simulink model "Main"  (Simulink 7.5)
settings: Solver=FixedStepDiscrete  StartTime=0.0  StopTime=Inf  FixedStep=0.001  RelTol=1e-3
undefined symbols (not defined in the file or in its folder): ecan1_buffered_transmit_matlab, ecan1_error_status_matlab, ecan1_init, ecan1_receive_matlab, u1, y1
libraries: simulink x20, dsPICdrivers x8
CloseFcn:
  | rtwprivate ssgencode ModelCloseRequest Main
settings Model: Creator=bwmairs  LastModifiedBy=bwmairs
settings OptimizationCC: InlineParams=on  InitFltsAndDblsToZero=on  OptimizeModelRefInitCode=on  LifeSpan=1
settings DebuggingCC: SaveWithParameterizedLinksMsg=none  StrictBusMsg=Warning
settings HardwareCC: ProdBitPerInt=16  ProdEndianess=LittleEndian  ProdWordSize=16  ProdHWDeviceType=16-bit Generic  TargetHWDeviceType=32-bit Generic
settings RTWCC: SystemTargetFile=dspic.tlc  TemplateMakefile=dspic_pic30_gcc.tmf  PostCodeGenCommand=dsPIC_Compile()  Description=Embedded Target for Microchip dsPIC (real-time)  ProcessScript=dspic_make_rtw_hook
settings RTWCC: CustomSource=|
  | ../../cBuffer.c
  | ../../ecanFunctions.c
  | ../../sbrk.c
settings CodeAppCC: IgnoreCustomStorageClasses=off
settings STFCustomTargetCC: TargetFcnLib=ansi_tfl_tmw.mat  IncludeMdlTerminateFcn=off  CombineOutputUpdateFcns=on  SuppressErrorStatus=on  ERTCustomFileBanners=on  SupportContinuousTime=off  SupportNonInlinedSFcns=off  CPPClassGenCompliant=on  SystemTargetFile=dspic.tlc
settings ERTTargetCC: TargetFcnLib=ansi_tfl_tmw.mat  MultiwordLength=2048  ParMdlRefBuildCompliant=off  CompOptLevelCompliant=off  IncludeMdlTerminateFcn=off  SuppressErrorStatus=on  ERTFirstTimeCompliant=off  ModelStepFunctionPrototypeControlCompliant=off  ExtModeMexFile=noextcomm  InlinedParameterPlacement=NonHierarchical  ERTSrcFileBannerTemplate=dsPIC_code_template.cgt  ERTHdrFileBannerTemplate=dsPIC_code_template.cgt  ERTDataSrcFileTemplate=dsPIC_code_template.cgt  ERTDataHdrFileTemplate=dsPIC_code_template.cgt  ERTCustomFileTemplate=dsPIC_main.tlc  ConvertIfToSwitch=off
settings CustomProperty: DataType=string  Value=C:\PROGRA~1\MATLAB\R2010a\bin\win32\gmake

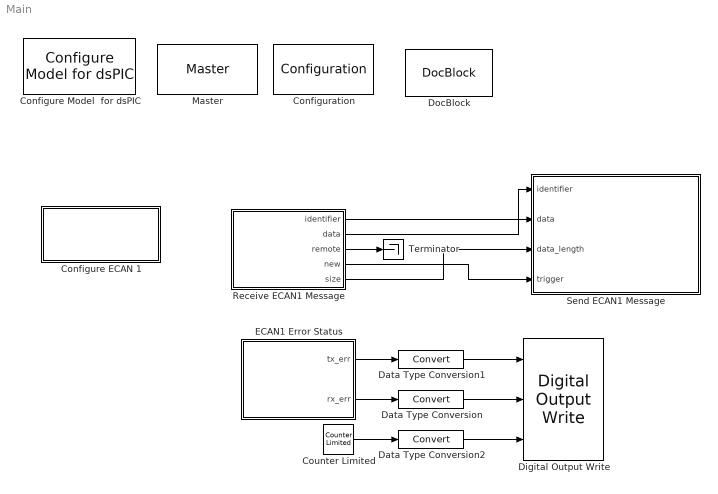
== system Main ==
  Configuration : dsPICdrivers/Configuration  SystemSampleTime=-1  double64=off
  Configure ECAN 1 : Subsystem  mask(Initialize ECAN 1){frame_setting=off, mode=Normal, dma_rx_chan=2, dma_tx_chan=0, baud=250000, ps1=8, pd=5, ps2=6, sjw=4, tq=20, triple_sample=on, dma_buf_size=4 buffers, rx_bufs=[1], tx_bufs=[0], buf_0_tx_pri=Highest, buf_0_rte=No, buf_1_tx_pri=Highest, buf_1_rte=No, buf_2_tx_pri=Lowest, buf_2_rte=No, buf_3_tx_pri=Lowest, buf_3_rte=No, buf_4_tx_pri=Lowest, buf_4_rte=No, buf_5_tx_pri=Lowest, buf_5_rte=No, buf_6_tx_pri=Lowest, buf_6_rte=No, buf_7_tx_pri=Lowest, buf_7_rte=No, mask_0=0, mask_0_mide=Match std or ext, mask_1=0, mask_1_mide=Match std or ext, mask_2=0, mask_2_mide=Match std or ext, filters=[0 1 2], filter_0=hex2dec('400'), filter_0_mask=0, filter_0_exide=Match only standard, filter_0_buf=1, filter_1=hex2dec('401'), filter_1_mask=0, filter_1_exide=Match only standard, filter_1_buf=1, filter_2=hex2dec('402'), filter_2_mask=0, filter_2_exide=Match only standard, filter_2_buf=1, filter_3=0, filter_3_mask=0, filter_3_exide=Match only standard, filter_3_buf=0, filter_4=0, filter_4_mask=0, filter_4_exide=Match only standard, filter_4_buf=0, filter_5=0, filter_5_mask=0, filter_5_exide=Match only standard, filter_5_buf=0, filter_6=0, filter_6_mask=0, filter_6_exide=Match only standard, filter_6_buf=0, filter_7=0, filter_7_mask=0, filter_7_exide=Match only standard, filter_7_buf=0, filter_8=0, filter_8_mask=0, filter_8_exide=Match only standard, filter_8_buf=0, filter_9=0, filter_9_mask=<empty>, filter_9_exide=Match only standard, filter_9_buf=0, filter_10=0, filter_10_mask=0, filter_10_exide=Match only standard, filter_10_buf=0, filter_11=0, filter_11_mask=0, filter_11_exide=Match only standard, filter_11_buf=0, filter_12=0, filter_12_mask=0, filter_12_exide=Match only standard, filter_12_buf=0, filter_13=0, filter_13_mask=0, filter_13_exide=Match only standard, filter_13_buf=0, filter_14=0, filter_14_mask=0, filter_14_exide=Match only standard, filter_14_buf=0, filter_15=0, filter_15_mask=0, filter_15_exide=Match only standard, filter_15_buf=0}
      mask prompts: frame_setting "Extended Frames (Standard if unchecked)"; dma_rx_chan "DMA Reception Channel"; dma_tx_chan "DMA Transmission Channel"; baud "Baud Rate (bps)"; ps1 "Phase Segment 1"; pd "Propagation Delay"; ps2 "Phase Segment 2"; sjw "Sync Jump Width"; tq "Time Quanta"; triple_sample "Triple-sample"; dma_buf_size "DMA Buffer Size"; rx_bufs "Reception Buffers"; tx_bufs "Transmission Buffers"; buf_0_tx_pri "Buffer 0 Transmission Priority"; buf_0_rte "Buffer 0 Remote Transmit Enable"; buf_1_tx_pri "Buffer 1 Transmission Priority"; buf_1_rte "Buffer 1 Remote Transmit Enable"; buf_2_tx_pri "Buffer 2 Transmission Priority"; buf_2_rte "Buffer 2 Remote Transmit Enable"; buf_3_tx_pri "Buffer 3 Transmission Priority"; buf_3_rte "Buffer 3 Remote Transmit Enable"; buf_4_tx_pri "Buffer 4 Transmission Priority"; buf_4_rte "Buffer 4 Remote Transmit Enable"; buf_5_tx_pri "Buffer 5 Transmission Priority"; buf_5_rte "Buffer 5 Remote Transmit Enable"; buf_6_tx_pri "Buffer 6 Transmission Priority"; buf_6_rte "Buffer 6 Remote Transmit Enable"; buf_7_tx_pri "Buffer 7 Transmission Priority"; buf_7_rte "Buffer 7 Remote Transmit Enable"; mask_0 "Mask 0"; mask_0_mide "Mask 0 Receive Mode"; mask_1 "Mask 1"; mask_1_mide "Mask 1 Receive Mode"; mask_2 "Mask 2"; mask_2_mide "Mask 2 Receive Mode"; filter_0 "Filter 0"; filter_0_mask "Filter 0 Mask"; filter_0_exide "Filter 0 Mode"; filter_0_buf "Filter 0 Buffer"; filter_1 "Filter 1"; filter_1_mask "Filter 1 Mask"; filter_1_exide "Filter 1 Mode"; filter_1_buf "Filter 1 Buffer"; filter_2 "Filter 2"; filter_2_mask "Filter 2 Mask"; filter_2_exide "Filter 2 Mode"; filter_2_buf "Filter 2 Buffer"; filter_3 "Filter 3"; filter_3_mask "Filter 3 Mask"; filter_3_exide "Filter 3 Mode"; filter_3_buf "Filter 3 Buffer"; filter_4 "Filter 4"; filter_4_mask "Filter 4 Mask"; filter_4_exide "Filter 4 Mode"; filter_4_buf "Filter 4 Buffer"; filter_5 "Filter 5"; filter_5_mask "Filter 5 Mask"; filter_5_exide "Filter 5 Mode"; filter_5_buf "Filter 5 Buffer"; filter_6 "Filter 6"; filter_6_mask "Filter 6 Mask"; filter_6_exide "Filter 6 Mode"; filter_6_buf "Filter 6 Buffer"; filter_7 "Filter 7"; filter_7_mask "Filter 7 Mask"; filter_7_exide "Filter 7 Mode"; filter_7_buf "Filter 7 Buffer"; filter_8 "Filter 8"; filter_8_mask "Filter 8 Mask"; filter_8_exide "Filter 8 Mode"; filter_8_buf "Filter 8 Buffer"; filter_9 "Filter 9"; filter_9_mask "Filter 9 Mask"; filter_9_exide "Filter 9 Mode"; filter_9_buf "Filter 9 Buffer"; filter_10 "Filter 10"; filter_10_mask "Filter 10 Mask"; filter_10_exide "Filter 10 Mode"; filter_10_buf "Filter 10 Buffer"; filter_11 "Filter 11"; filter_11_mask "Filter 11 Mask"; filter_11_exide "Filter 11 Mode"; filter_11_buf "Filter 11 Buffer"; filter_12 "Filter 12"; filter_12_mask "Filter 12 Mask"; filter_12_exide "Filter 12 Mode"; filter_12_buf "Filter 12 Buffer"; filter_13 "Filter 13"; filter_13_mask "Filter 13 Mask"; filter_13_exide "Filter 13 Mode"; filter_13_buf "Filter 13 Buffer"; filter_14 "Filter 14"; filter_14_mask "Filter 14 Mask"; filter_14_exide "Filter 14 Mode"; filter_14_buf "Filter 14 Buffer"; filter_15 "Filter 15"; filter_15_mask "Filter 15 Mask"; filter_15_exide "Filter 15 Mode"; filter_15_buf "Filter 15 Buffer"
      mask help: Initializes the ECAN 1 module on the dsPIC33f. Allows for configuration of almost all ECAN options to produce a usable system.
      mask init:
      | parameters = uint16(zeros(53,1));
      | 
      | %% Generate parameter 1
      | parameters(1) = frame_setting;
      | mode_id = 0;
      | switch mode
      |     case 'Disabled'
      |         mode_id = 1;
      |     case 'Loopback'
      |         mode_id = 2;
      |     case 'Listen only'
      |         mode_id = 3;
      |     case 'Listen all'
      |         mode_id = 7;
      | end
      | parameters(1) = bitor(parameters(1), bitshift(mode_id, 2));
      | parameters(1) = bitor(parameters(1), bitshift(dma_rx_chan, 5));
      | parameters(1) = bitor(parameters(1), bitshift(dma_tx_chan, 8));
      | 
      | %% Generate parameter 2
      | parameters(2) = baud / 100;
      | 
      | %% Generate parameter 3
      | h = find_system(bdroot(gcb),'FollowLinks','on','LookUnderMasks','all','Tag','dsPIC_MASTER');
      | fcy = 0;
      | if ~isempty(h)
      |     %OverrideFcy = strcmp(get_param(h{1},'OverrideFcy'),'on');
      |     %if (OverrideFcy == 1)
      |     %    fcy = str2num(get_param(h{1},'NewFcy'));     %% overridded fcy
      |     %else
      |         fcy = str2num(get_param(h{1},'fcy'));
      |     %end 
      | end
      | parameters(3) = fcy / 1000;
      | 
      | %% Generate parameter 4
      | parameters(4) = ps1 - 1;
      | parameters(4) = bitor(parameters(4), bitshift(pd - 1, 3));
      | parameters(4) = bitor(parameters(4), bitshift(ps2 - 1, 6));
      | parameters(4) = bitor(parameters(4), bitshift(sjw - 1, 9));
      | if triple_sample == 1
      |     parameters(4) = bitset(parameters(4),12);
      | end
      | 
      | %% Generate parameter 5
      | for k = 1:length(filters)
      |     parameters(5) = bitset(parameters(5),filters(k)+1);
      | end;
      | 
      | % Map filter mask values into proper values
      | filter_masks = [filter_0_mask; filter_1_mask; filter_2_mask; filter_3_mask; filter_4_mask; filter_5_mask; filter_6_mask; filter_7_mask; filter_8_mask; filter_9_mask; filter_10_mask; filter_11_mask; filter_12_mask; filter_13_mask; filter_14_mask; filter_15_mask;];
      | filter_masks = filter_masks - 2;
      | filter_masks(filter_masks == -1) = 3;
      | 
      | %% Generate parameters 6 and 7
      | for k = 1:length(filters);
      |     filter = filters(k) + 1;
      |     if filter < 9
      |         parameters(6) = bitor(parameters(6), bitshift(filter_masks(filter),2*(filter-1)));
      |     else
      |         parameters(7) = bitor(parameters(7), bitshift(filter_masks(filter),2*(filter-9)));
      |     end
      | end
      | 
      | % Generate parameters 8 and 9
      | parameters(8) = bitshift(bitand(mask_0,hex2dec('18000000')),-27); % EID17-16
      | parameters(8) = bitor(parameters(8), bitshift(bitand(mask_0,hex2dec('7FF')), 5)); % SID
      | parameters(8) = bitor(parameters(8), bitshift(mask_0_mide - 1, 3)); % MIDE
      | parameters(9) = bitshift(bitand(mask_0,hex2dec('7FFF800')),-11); % EID15-0
      | 
      | %% Generate parameters 10 and 11
      | parameters(10) = bitshift(bitand(mask_1,hex2dec('18000000')),-27); % EID17-16
      | parameters(10) = bitor(parameters(10), bitshift(bitand(mask_1,hex2dec('7FF')), 5)); % SID
      | parameters(10) = bitor(parameters(10), bitshift(mask_1_mide - 1, 3)); % MIDE
      | parameters(11) = bitshift(bitand(mask_1,hex2dec('7FFF800')),-11); % EID15-0
      | 
      | %% Generate parameters 12 and 13
      | parameters(12) = bitshift(bitand(mask_2,hex2dec('18000000')),-27); % EID17-16
      | parameters(12) = bitor(parameters(12), bitshift(bitand(mask_2,hex2dec('7FF')), 5)); % SID
      | parameters(12) = bitor(parameters(12), bitshift(mask_2_mide - 1, 3)); % MIDE
      | parameters(13) = bitshift(bitand(mask_2,hex2dec('7FFF800')),-11); % EID15-0
      | 
      | % Generate parameters 14-17
      | buf_priorities = [buf_0_tx_pri;buf_1_tx_pri;buf_2_tx_pri;buf_3_tx_pri;buf_4_tx_pri;buf_5_tx_pri;buf_6_tx_pri;buf_7_tx_pri] - 1;
      | buf_rtes = [buf_0_rte;buf_1_rte;buf_2_rte;buf_3_rte;buf_4_rte;buf_5_rte;buf_6_rte;buf_7_rte] - 1;
      | 
      | % Create a vector of chars to modify
      | regs = uint16(zeros(8,1));
      | 
      | % Go through all enabled transmission buffers setting appropriate bits
      | for b = 1:size(tx_bufs,1)
      |     
      |     index = tx_bufs(b) + 1;
      |     
      |     % Set transmission bit
      |     regs(index) = bitset(regs(index),8);
      | 
      |     % Set priority bits
      |     regs(index) = bitor(regs(index), buf_priorities(index));
      | 
      |     % Set remote transmit enable bits
      |     if buf_rtes(index) == 1
      |         regs(index) = bitset(regs(index),3);
      |     end
      | end
      | 
      | for b = 1:size(rx_bufs,1)
      |     
      |     index = rx_bufs(b) + 1;
      | 
      |     % Set priority bits
      |     regs(index) = bitor(regs(index), buf_priorities(index));
      | 
      |     % Set remote transmit enable bits
      |     if buf_rtes(index) == 1
      |         regs(index) = bitset(regs(index),3);
      |     end
      | end
      | 
      | % Map our matrix into registers
      | parameters(14) = bitor(bitshift(regs(2),8), regs(1));
      | parameters(15) = bitor(bitshift(regs(4),8), regs(3));
      | parameters(16) = bitor(bitshift(regs(6),8), regs(5));
      | parameters(17) = bitor(bitshift(regs(8),8), regs(7));
      | 
      | % Map the filter buffer values to corresponding bit values
      | filter_buffers = [filter_0_buf; filter_1_buf; filter_2_buf; filter_3_buf; filter_4_buf; filter_5_buf; filter_6_buf; filter_7_buf; filter_8_buf; filter_9_buf; filter_10_buf; filter_11_buf; filter_12_buf; filter_13_buf; filter_14_buf; filter_15_buf;];
      | filter_buffers = filter_buffers - 1;
      | 
      | %% Generate parameter 18
      | if bitget(parameters(5),1) == 1
      |     parameters(18) = filter_buffers(1);
      | end
      | if bitget(parameters(5),2) == 1
      |     parameters(18) = bitor(parameters(18), bitshift(filter_buffers(2), 4));
      | end
      | if bitget(parameters(5),3) == 1
      |     parameters(18) = bitor(parameters(18), bitshift(filter_buffers(3), 8));
      | end
      | if bitget(parameters(5),4) == 1
      |     parameters(18) = bitor(parameters(18), bitshift(filter_buffers(4), 12));
      | end
      | 
      | %% Generate parameter 19
      | if bitget(parameters(5),5) == 1
      |     parameters(19) = filter_buffers(5);
      | end
      | if bitget(parameters(5),6) == 1
      |     parameters(19) = bitor(parameters(19), bitshift(filter_buffers(6), 4));
      | end
      | if bitget(parameters(5),7) == 1
      |     parameters(19) = bitor(parameters(19), bitshift(filter_buffers(7), 8));
      | end
      | if bitget(parameters(5),8) == 1
      |     parameters(19) = bitor(parameters(19), bitshift(filter_buffers(8), 12));
      | end
      | 
      | %% Generate parameter 20
      | if bitget(parameters(5),9) == 1
      |     parameters(20) = filter_buffers(9);
      | end
      | if bitget(parameters(5),10) == 1
      |     parameters(20) = bitor(parameters(20), bitshift(filter_buffers(10), 4));
      | end
      | if bitget(parameters(5),11) == 1
      |     parameters(20) = bitor(parameters(20), bitshift(filter_buffers(11), 8));
      | end
      | if bitget(parameters(5),12) == 1
      |     parameters(20) = bitor(parameters(20), bitshift(filter_buffers(12), 12));
      | end
      | 
      | %% Generate parameter 21
      | if bitget(parameters(5),13) == 1
      |     parameters(21) = filter_buffers(13);
      | end
      | if bitget(parameters(5),14) == 1
      |     parameters(21) = bitor(parameters(21), bitshift(filter_buffers(14), 4));
      | end
      | if bitget(parameters(5),15) == 1
      |     parameters(21) = bitor(parameters(21), bitshift(filter_buffers(15), 8));
      | end
      | if bitget(parameters(5),16) == 1
      |     parameters(21) = bitor(parameters(21), bitshift(filter_buffers(16), 12));
      | end
      | 
      | % Generate parameters 22 and 23
      | parameters(22) = bitshift(bitand(filter_0,hex2dec('18000000')),-27); % EID17-16
      | parameters(22) = bitor(parameters(22), bitshift(bitand(filter_0,hex2dec('7FF')), 5)); % SID
      | parameters(22) = bitor(parameters(22), bitshift(filter_0_exide - 1, 3)); % EXIDE
      | parameters(23) = bitshift(bitand(uint32(filter_0),hex2dec('7FFF800')),-11); % EID15-0
      | 
      | %% Generate parameters 24 and 25
      | parameters(24) = bitshift(bitand(filter_1,hex2dec('18000000')),-27); % EID17-16
      | parameters(24) = bitor(parameters(24), bitshift(bitand(filter_1,hex2dec('7FF')), 5)); % SID
      | parameters(24) = bitor(parameters(24), bitshift(filter_1_exide - 1, 3)); % EXIDE
      | parameters(25) = bitshift(bitand(uint32(filter_1),hex2dec('7FFF800')),-11); % EID15-0
      | 
      | %% Generate parameters 26 and 27
      | parameters(26) = bitshift(bitand(filter_2,hex2dec('18000000')),-27); % EID17-16
      | parameters(26) = bitor(parameters(26), bitshift(bitand(filter_2,hex2dec('7FF')), 5)); % SID
      | parameters(26) = bitor(parameters(26), bitshift(filter_2_exide - 1, 3)); % EXIDE
      | parameters(27) = bitshift(bitand(uint32(filter_2),hex2dec('7FFF800')),-11); % EID15-0
      | 
      | %% Generate parameters 28 and 29
      | parameters(28) = bitshift(bitand(filter_3,hex2dec('18000000')),-27); % EID17-16
      | parameters(28) = bitor(parameters(28), bitshift(bitand(filter_3,hex2dec('7FF')), 5)); % SID
      | parameters(28) = bitor(parameters(28), bitshift(filter_3_exide - 1, 3)); % EXIDE
      | parameters(29) = bitshift(bitand(uint32(filter_3),hex2dec('7FFF800')),-11); % EID15-0
      | 
      | %% Generate parameters 30 and 31
      | parameters(30) = bitshift(bitand(filter_4,hex2dec('18000000')),-27); % EID17-16
      | parameters(30) = bitor(parameters(30), bitshift(bitand(filter_4,hex2dec('7FF')), 5)); % SID
      | parameters(30) = bitor(parameters(30), bitshift(filter_4_exide - 1, 3)); % EXIDE
      | parameters(31) = bitshift(bitand(uint32(filter_4),hex2dec('7FFF800')),-11); % EID15-0
      | 
      | %% Generate parameters 32 and 33
      | parameters(32) = bitshift(bitand(filter_5,hex2dec('18000000')),-27); % EID17-16
      | parameters(32) = bitor(parameters(32), bitshift(bitand(filter_5,hex2dec('7FF')), 5)); % SID
      | parameters(32) = bitor(parameters(32), bitshift(filter_5_exide - 1, 3)); % EXIDE
      | parameters(33) = bitshift(bitand(uint32(filter_5),hex2dec('7FFF800')),-11); % EID15-0
      | 
      | %% Generate parameters 34 and 35
      | parameters(34) = bitshift(bitand(filter_6,hex2dec('18000000')),-27); % EID17-16
      | parameters(34) = bitor(parameters(34), bitshift(bitand(filter_6,hex2dec('7FF')), 5)); % SID
      | parameters(34) = bitor(parameters(34), bitshift(filter_6_exide - 1, 3)); % EXIDE
      | parameters(35) = bitshift(bitand(uint32(filter_6),hex2dec('7FFF800')),-11); % EID15-0
      | 
      | %% Generate parameters 36 and 37
      | parameters(36) = bitshift(bitand(filter_7,hex2dec('18000000')),-27); % EID17-16
      | parameters(36) = bitor(parameters(36), bitshift(bitand(filter_7,hex2dec('7FF')), 5)); % SID
      | parameters(36) = bitor(parameters(36), bitshift(filter_7_exide - 1, 3)); % EXIDE
      | parameters(37) = bitshift(bitand(uint32(filter_7),hex2dec('7FFF800')),-11); % EID15-0
      | 
      | %% Generate parameters 38 and 39
      | parameters(38) = bitshift(bitand(filter_8,hex2dec('18000000')),-27); % EID17-16
      | parameters(38) = bitor(parameters(38), bitshift(bitand(filter_8,hex2dec('7FF')), 5)); % SID
      | parameters(38) = bitor(parameters(38), bitshift(filter_8_exide - 1, 3)); % EXIDE
      | parameters(39) = bitshift(bitand(uint32(filter_8),hex2dec('7FFF800')),-11); % EID15-0
      | 
      | %% Generate parameters 40 and 41
      | parameters(40) = bitshift(bitand(filter_9,hex2dec('18000000')),-27); % EID17-16
      | parameters(40) = bitor(parameters(40), bitshift(bitand(filter_9,hex2dec('7FF')), 5)); % SID
      | parameters(40) = bitor(parameters(40), bitshift(filter_9_exide - 1, 3)); % EXIDE
      | parameters(41) = bitshift(bitand(uint32(filter_9),hex2dec('7FFF800')),-11); % EID15-0
      | 
      | %% Generate parameters 42 and 43
      | parameters(42) = bitshift(bitand(filter_10,hex2dec('18000000')),-27); % EID17-16
      | parameters(42) = bitor(parameters(42), bitshift(bitand(filter_10,hex2dec('7FF')), 5)); % SID
      | parameters(42) = bitor(parameters(42), bitshift(filter_10_exide - 1, 3)); % EXIDE
      | parameters(43) = bitshift(bitand(uint32(filter_10),hex2dec('7FFF800')),-11); % EID15-0
      | 
      | %% Generate parameters 44 and 45
      | parameters(44) = bitshift(bitand(filter_11,hex2dec('18000000')),-27); % EID17-16
      | parameters(44) = bitor(parameters(44), bitshift(bitand(filter_11,hex2dec('7FF')), 5)); % SID
      | parameters(44) = bitor(parameters(44), bitshift(filter_11_exide - 1, 3)); % EXIDE
      | parameters(45) = bitshift(bitand(uint32(filter_11),hex2dec('7FFF800')),-11); % EID15-0
      | 
      | %% Generate parameters 46 and 47
      | parameters(46) = bitshift(bitand(filter_12,hex2dec('18000000')),-27); % EID17-16
      | parameters(46) = bitor(parameters(46), bitshift(bitand(filter_12,hex2dec('7FF')), 5)); % SID
      | parameters(46) = bitor(parameters(46), bitshift(filter_12_exide - 1, 3)); % EXIDE
      | parameters(47) = bitshift(bitand(uint32(filter_12),hex2dec('7FFF800')),-11); % EID15-0
      | 
      | %% Generate parameters 48 and 49
      | parameters(48) = bitshift(bitand(filter_13,hex2dec('18000000')),-27); % EID17-16
      | parameters(48) = bitor(parameters(48), bitshift(bitand(filter_13,hex2dec('7FF')), 5)); % SID
      | parameters(48) = bitor(parameters(48), bitshift(filter_13_exide - 1, 3)); % EXIDE
      | parameters(49) = bitshift(bitand(uint32(filter_13),hex2dec('7FFF800')),-11); % EID15-0
      | 
      | %% Generate parameters 50 and 51
      | parameters(50) = bitshift(bitand(filter_14,hex2dec('18000000')),-27); % EID17-16
      | parameters(50) = bitor(parameters(50), bitshift(bitand(filter_14,hex2dec('7FF')), 5)); % SID
      | parameters(50) = bitor(parameters(50), bitshift(filter_14_exide - 1, 3)); % EXIDE
      | parameters(51) = bitshift(bitand(uint32(filter_14),hex2dec('7FFF800')),-11); % EID15-0
      | 
      | %% Generate parameters 52 and 53
      | parameters(52) = bitshift(bitand(filter_15,hex2dec('18000000')),-27); % EID17-16
      | parameters(52) = bitor(parameters(52), bitshift(bitand(filter_15,hex2dec('7FF')), 5)); % SID
      | parameters(52) = bitor(parameters(52), bitshift(filter_15_exide - 1, 3)); % EXIDE
      | parameters(53) = bitshift(bitand(uint32(filter_15),hex2dec('7FFF800')),-11); % EID15-0
      mask StyleString: checkbox,popup(Disabled|Listen all|Listen only|Loopback|Normal),edit,edit,edit,edit,edit,edit,popup(1|2|3|4),edit,checkbox,popup(4 buffers|6 buffers|8 buffers|12 buffers|16 buffers|24 buffers|32 buffers),edit,edit,popup(Lowest|Low|High|Highest),popup(No|Yes),popup(Lowest|Low|High|Highest),popup(No|Yes),popup(Lowest|Low|High|Highest),popup(No|Yes),popup(Lowest|Low|High|Highest),popup(No|Yes),popup(Lowest|Low|High|Highest),popup(No|Yes),popup(Lowest|Low|High|Highest),popup(No|Yes),popup(Lowest|Low|High|Highest),popup(No|Yes),popup(Lowest|Low|High|Highest),popup(No|Yes),edit,popup(Match std or ext|Obey filter mode),edit,popup(Match std or ext|Obey filter mode),edit,popup(Match std or ext|Obey filter mode),edit,edit,popup(--|0|1|2),popup(Match only standard|Match only extended),popup(0|1|2|3|4|5|6|7|8|9|10|11|12|13|14|FIFO),edit,popup(--|0|1|2),popup(Match only standard|Match only extended),popup(0|1|2|3|4|5|6|7|8|9|10|11|12|13|14|FIFO),edit,popup(--|0|1|2),popup(Match only standard|Match only extended),popup(0|1|2|3|4|5|6|7|8|9|10|11|12|13|14|FIFO),edit,popup(--|0|1|2),popup(Match only standard|Match only extended),popup(0|1|2|3|4|5|6|7|8|9|10|11|12|13|14|FIFO),edit,popup(--|0|1|2),popup(Match only standard|Match only extended),popup(0|1|2|3|4|5|6|7|8|9|10|11|12|13|14|FIFO),edit,popup(--|0|1|2),popup(Match only standard|Match only extended),popup(0|1|2|3|4|5|6|7|8|9|10|11|12|13|14|FIFO),edit,popup(--|0|1|2),popup(Match only standard|Match only extended),popup(0|1|2|3|4|5|6|7|8|9|10|11|12|13|14|FIFO),edit,popup(--|0|1|2),popup(Match only standard|Match only extended),popup(0|1|2|3|4|5|6|7|8|9|10|11|12|13|14|FIFO),edit,popup(--|0|1|2),popup(Match only standard|Match only extended),popup(0|1|2|3|4|5|6|7|8|9|10|11|12|13|14|FIFO),edit,popup(<empty>),popup(Match only standard|Match only extended),popup(0|1|2|3|4|5|6|7|8|9|10|11|12|13|14|FIFO),edit,popup(--|0|1|2),popup(Match only standard|Match only extended),popup(0|1|2|3|4|5|6|7|8|9|10|11|12|13|14|FIFO),edit,popup(--|0|1|2),popup(Match only standard|Match only extended),popup(0|1|2|3|4|5|6|7|8|9|10|11|12|13|14|FIFO),edit,popup(--|0|1|2),popup(Match only standard|Match only extended),popup(0|1|2|3|4|5|6|7|8|9|10|11|12|13|14|FIFO),edit,popup(--|0|1|2),popup(Match only standard|Match only extended),popup(0|1|2|3|4|5|6|7|8|9|10|11|12|13|14|FIFO),edit,popup(--|0|1|2),popup(Match only standard|Match only extended),popup(0|1|2|3|4|5|6|7|8|9|10|11|12|13|14|FIFO),edit,popup(--|0|1|2),popup(Match only standard|Match only extended),popup(0|1|2|3|4|5|6|7|8|9|10|11|12|13|14|FIFO)
      mask CallbackString:
      | |||||tq = 1 + str2num(get_param(gcb, 'ps1')) + str2num(get_param(gcb, 'pd')) + str2num(get_param(gcb, 'ps2'));
      | set_param(gcb, 'tq', int2str(tq));|tq = 1 + str2num(get_param(gcb, 'ps1')) + str2num(get_param(gcb, 'pd')) + str2num(get_param(gcb, 'ps2'));
      | set_param(gcb, 'tq', int2str(tq));|tq = 1 + str2num(get_param(gcb, 'ps1')) + str2num(get_param(gcb, 'pd')) + str2num(get_param(gcb, 'ps2'));
      | set_param(gcb, 'tq', int2str(tq));||||||filters = eval(get_param(gcb,'tx_bufs'));
      | mVisibilities = get_param(gcb,'MaskVisibilities');
      | mNames = get_param(gcb,'MaskNames');
      | for i = 1:size(mNames);
      | 	n = mNames{i};
      |     if size(n,2) > 4 && strcmp(n(1:4), 'buf_') == 1
      |         filterNumber = sscanf(n, 'buf_%d');
      |         if isempty(find(filters == filterNumber, 1)) == 0
      |              mVisibilities{i} = 'on';
      |         else
      |              mVisibilities{i} = 'off';
      |         end
      |     end
      | end
      | set_param(gcb, 'MaskVisibilities', mVisibilities);|||||||||||||||||||||||filters = eval(get_param(gcb,'filters'));
      | mVisibilities = get_param(gcb,'MaskVisibilities');
      | mNames = get_param(gcb,'MaskNames');
      | for i = 1:size(mNames);
      | 	n = mNames{i};
      |     if size(n,2) > 7 && strcmp(n(1:7), 'filter_') == 1
      |         filterNumber = sscanf(n, 'filter_%d');
      |         if isempty(find(filters == filterNumber, 1)) == 0
      |              mVisibilities{i} = 'on';
      |         else
      |              mVisibilities{i} = 'off';
      |         end
      |     end
      | end
      | set_param(gcb, 'MaskVisibilities', mVisibilities);||||||||||||||||||||||||||||||||||||||||||||||||||||||||||||||||
      mask Display: text(0.5,0.5,'Configure ECAN1','horizontalAlignment','center','verticalAlignment','middle');
  Configure Model  for dsPIC : dsPICdrivers/Simulink Configuration/Configure Model  for dsPIC
  Counter Limited : simulink/Sources/Counter Limited  SystemSampleTime=-1  uplimit=1  tsamp=.1
  Data Type Conversion : DataTypeConversion  OutDataType=sfix(16)  OutScaling=2^0
  Data Type Conversion1 : DataTypeConversion  OutDataType=sfix(16)  OutScaling=2^0
  Data Type Conversion2 : DataTypeConversion  OutDataType=sfix(16)  OutScaling=2^0
  Digital Output Write : dsPICdrivers/Digital I//O/Digital Output Write  Tag=dsPIC_Digital_Output  Priority=5  PORT=A  Pin=[0 1 7]  Simultaneous=off  OrderingInOutPopup=None
  DocBlock : simulink/Model-Wide Utilities/DocBlock  SystemSampleTime=-1  DocumentType=Text
      content=|
      | This model recreates the Crosswire application note from Microchip.
      | The Debugging directory includes an MPLAB project that can compile and load
      | the MATLAB-generated code in order to facilitate debugging.
  ECAN1 Error Status : Subsystem  mask(ECAN 1 Reception Block){ecan1_error_sample_time=.1}
      mask prompts: ecan1_error_sample_time "Sampling time"
      mask help:
      | This block will receive CAN messages over the ECAN1 peripheral on the dsPIC33f.
      | Outputs:
      | identifier - uint32 containing SID and EID
      | data - Variable-sized array (between 0 and 8) of uint8s
      | remote - boolean value specifying if this is a remote transmit request
      mask Display: disp('ECAN1 ERR');
  Master : dsPICdrivers/Master  Tag=dsPIC_MASTER  Priority=1  TimeStepType=Timer1  picType=choose_dsPIC_Target  fcy=5e6  Quartz_33f=5e6  PLLActive_33f=off  fcyDesired_33f=0  tmr1="[1  4999  0]"  tmr1Info="Time Step : 0.001  ;   Error : 0%  PR1=4999"  tmr2345="[0  0  0  0  0  0  0  0]"  tmr2345cfg=[-1 -1 -1 -1 -1 -1 -1 -1]  IOautoConf=on  typePort="[ 10  10   0   0   0   0   0  10   0   0   0   0   0   0   0   0   0   0   0   0   0   0   0   0   0   0   0   0   0   0   0   0   0   0   0   0   0   0   0   0   0   0   0   0   0   0   0   0   0   0   0   0   0   0   0   0   0   0   0   0   0   0   0   0   0   0   0   0   0   0   0   0   0   0   0   0   0   0   0   0   0   0   0   0   0   0   0   0   0   0   0   0   0   0   0   0   0   0   0   0   0   0   0   0   0   0   0   0   0   0   0   0 ]"  TRIS="[ 65404  65535  65535  65535  65535  65535  65535 ]"  ADPCFG=131  MasterBusyPort=None  MasterOverloadPort=None  FOSC=CSW_FSCM_OFF  ClockSwitchMonitor=Both disabled  TempProtection_33f=TEMP_ON  FPBOR=PBOR_OFF  PWRT=PWRT_OFF  MCLR=MCLR_DIS  ICD=ICS_NONE  JTAGEN=JTAGEN_OFF  PowerSave=off  OverrideFcy=off  NewFcy=1e6  PR2345="[65535  65535  65535  65535  65535  65535  65535  65535]"
  Receive ECAN1 Message : Subsystem  mask(ECAN 1 Reception Block){ecan1_receive_sample_time=.01}
      mask prompts: ecan1_receive_sample_time "Sampling time"
      mask help:
      | This block will receive CAN messages over the ECAN1 peripheral on the dsPIC33f.
      | Outputs:
      | identifier - uint32 containing SID and EID
      | data - Variable-sized array (between 0 and 8) of uint8s
      | remote - boolean value specifying if this is a remote transmit request
      mask Display: disp('ECAN1 RX');
  Send ECAN1 Message : Subsystem  Tag=dsPIC_MASTER  mask(Send ECAN Message){buffer=0, identifier=hex2dec('401'), identifier_from_input=on, ide=off, remote=off, data=[hex2dec('11') hex2dec('12') hex2dec('13') hex2dec('14')], data_length=4, data_from_input=on, c_func_sample_time=.01, trigger_on_input=on}
      mask prompts: identifier_from_input "Identifier from input"; data_length "Data length"; data_from_input "Data from input"; c_func_sample_time "Sample time"; trigger_on_input "Trigger on input"
      mask help: This block allows for the transmission of a message over the ECAN module.
      mask CallbackString:
      | ||mEnables = get_param(gcb,'MaskEnables');
      | enabled = get_param(gcb, 'identifier_from_input');
      | if strcmp(enabled,'on');
      |     replace_block([gcb '/identifier'],'Constant','Inport','noprompt');
      |     mEnables{2} = 'off';
      |     set_param([gcb '/identifier'],'Port','1');
      | else
      |     replace_block([gcb '/identifier'],'Inport','Constant','noprompt');
      |     mEnables{2} = 'on';
      |     set_param([gcb '/identifier'],'Value','identifier');
      | end
      | set_param(gcb, 'MaskEnables', mEnables);
      | |||data = eval(get_param(gcb, 'data'));
      | y = size(data,1);
      | x = size(data,2);
      | if y > 1 && x > 1
      |     error('Data must be a 1-dimensional vector')
      | else
      |     if or(x > 8, y > 8)
      |         error('Data cannot be larger than 8-bytes');
      |     end
      | end
      | 
      | set_param(gcb, 'data_length', num2str(length(data)));|data_length = eval(get_param(gcb, 'data_length'));
      | if or(data_length < 0, data_length > 9)
      |     error('Data cannot be more than 8 bytes or less than 0.')
      | end|mEnables = get_param(gcb,'MaskEnables');
      | enabled = get_param(gcb, 'data_from_input');
      | if strcmp(enabled,'on');
      |     replace_block([gcb '/data'],'Constant','Inport','noprompt');
      |     replace_block([gcb '/data_length'],'Constant','Inport','noprompt');
      |     mEnables{6} = 'off';
      |     mEnables{7} = 'off';
      |     port = 1;
      |     if ~isempty(find_system(gcb,'LookUnderMasks','all','Name','identifier'))
      |         port = 2;
      |     end
      |     set_param([gcb '/data'],'Port',num2str(port));
      |     set_param([gcb '/data_length'],'Port',num2str(port+1));
      | else
      |     replace_block([gcb '/data'],'Inport','Constant','noprompt');
      |     replace_block([gcb '/data_length'],'Inport','Constant','noprompt');
      |     mEnables{6} = 'on';
      |     mEnables{7} = 'on';
      |     set_param([gcb '/data'],'Value','data');
      |     set_param([gcb '/data'],'OutDataTypeMode','uint8');
      |     set_param([gcb '/data_length'],'Value','data_length');
      |     set_param([gcb '/data_length'],'OutDataTypeMode','uint8');
      | end
      | set_param(gcb, 'MaskEnables', mEnables);
      | ||mEnables = get_param(gcb,'MaskEnables');
      | enabled = get_param(gcb, 'trigger_on_input');
      | c_func_blk = find_system(gcb,'LookUnderMasks','all','FunctionName','dsPIC_C_function_Call');
      | if strcmp(enabled,'on');
      |     mEnables{9} = 'off';
      |     %set_param(c_func_blk,'SampleTime','-1');
      |     replace_block([gcb '/trigger'],'Constant','Inport','noprompt');
      | else
      |     mEnables{9} = 'on';
      |     %set_param(c_func_blk,'SampleTime','c_func_sample_time');
      |     replace_block([gcb '/trigger'],'Inport','Constant','noprompt');
      |     %set_param([gcb '/trigger'],'Value','1');
      | end
      | set_param(gcb, 'MaskEnables', mEnables);
      mask Display: disp('ECAN1 TX');
  Terminator : Terminator
  wires:
  Receive ECAN1 Message/3(remote) -> Terminator/1
  ECAN1 Error Status/2(rx_err) -> Data Type Conversion/1
  ECAN1 Error Status/1(tx_err) -> Data Type Conversion1/1
  Counter Limited/1 -> Data Type Conversion2/1
  Data Type Conversion1/1 -> Digital Output Write/1
  Data Type Conversion/1 -> Digital Output Write/2
  Data Type Conversion2/1 -> Digital Output Write/3
  Receive ECAN1 Message/2(data) -> Send ECAN1 Message/2(data)
  Receive ECAN1 Message/4(new) -> Send ECAN1 Message/4(trigger)
  Receive ECAN1 Message/5(size) -> Send ECAN1 Message/3(data_length)
  Receive ECAN1 Message/1(identifier) -> Send ECAN1 Message/1(identifier)

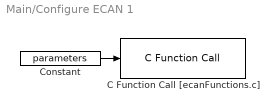
== system Main/Configure ECAN 1 ==
  C Function Call [ecanFunctions.c] : dsPICdrivers/OTHERS/C Function Call  Tag=dsPIC_dsPIC_CFunctionCall  fctName='ecan1_init'  INPUT_SIZE=53  INPUT1=uint16  INPUT2=--  INPUT3=--  OUTPUT_SIZE=1  OUTPUT1=--  SampleTime=Inf  InputType=[ 4 ]  OutputType=[ ]  FctDeclaration=extern void ecan1_init(uint16_T* u1);  FctCall=ecan1_init(*%u1);  OrderingInOutPopup=None
  Constant : Constant  Value=parameters  OutDataTypeMode=uint16  OutDataType=sfix(16)  OutScaling=2^0  OutDataTypeStr=uint16
  wires:
  Constant/1 -> C Function Call [ecanFunctions.c]/1

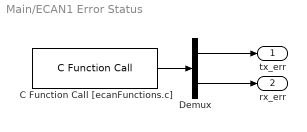
== system Main/ECAN1 Error Status ==
  C Function Call [ecanFunctions.c] : dsPICdrivers/OTHERS/C Function Call  Tag=dsPIC_dsPIC_CFunctionCall  fctName='ecan1_error_status_matlab'  INPUT_SIZE=1  INPUT1=--  INPUT2=--  INPUT3=--  OUTPUT_SIZE=2  OUTPUT1=uint8  SampleTime=ecan1_error_sample_time  InputType=[ ]  OutputType=[ 2 ]  FctDeclaration=extern void ecan1_error_status_matlab(uint8_T* y1);  FctCall=ecan1_error_status_matlab(*%y1);  OrderingInOutPopup=None
  Demux : Demux  Outputs=2
  tx_err : Outport  OutDataType=sfix(16)  OutScaling=2^0
  rx_err : Outport  Port=2  OutDataType=sfix(16)  OutScaling=2^0
  wires:
  Demux/2 -> rx_err/1
  Demux/1 -> tx_err/1
  C Function Call [ecanFunctions.c]/1 -> Demux/1

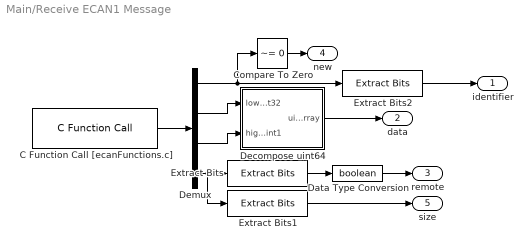
== system Main/Receive ECAN1 Message ==
  C Function Call [ecanFunctions.c] : dsPICdrivers/OTHERS/C Function Call  Tag=dsPIC_dsPIC_CFunctionCall  fctName='ecan1_receive_matlab'  INPUT_SIZE=1  INPUT1=--  INPUT2=--  INPUT3=--  OUTPUT_SIZE=4  OUTPUT1=uint32  SampleTime=ecan1_receive_sample_time  InputType=[ ]  OutputType=[ 6 ]  FctDeclaration=extern void ecan1_receive_matlab(uint32_T* y1);  FctCall=ecan1_receive_matlab(*%y1);  OrderingInOutPopup=None
  Compare To Zero : simulink/Logic and Bit Operations/Compare To Zero  SystemSampleTime=-1  relop=~=  LogicOutDataTypeMode=uint8  ZeroCross=off
  Data Type Conversion : DataTypeConversion  OutDataTypeMode=boolean  OutDataType=sfix(16)  OutScaling=2^0  OutDataTypeStr=boolean
  Decompose uint64 : Subsystem
  Demux : Demux
  Extract Bits : simulink/Logic and Bit Operations/Extract Bits  SystemSampleTime=-1  bitsToExtract=Lower half  numBits=8  bitIdxRange=[0 7]  outScalingMode=Treat bit field as an integer
  Extract Bits1 : simulink/Logic and Bit Operations/Extract Bits  SystemSampleTime=-1  bitsToExtract=Range of bits  numBits=8  bitIdxRange=[16 23]  outScalingMode=Treat bit field as an integer
  Extract Bits2 : simulink/Logic and Bit Operations/Extract Bits  SystemSampleTime=-1  bitsToExtract=Range ending with least significant bit  numBits=29  bitIdxRange=[0 7]  outScalingMode=Treat bit field as an integer
  identifier : Outport  OutDataType=sfix(16)  OutScaling=2^0
  data : Outport  Port=2  OutDataType=sfix(16)  OutScaling=2^0
  remote : Outport  Port=3  OutDataType=sfix(16)  OutScaling=2^0
  new : Outport  Port=4  OutDataType=sfix(16)  OutScaling=2^0
  size : Outport  Port=5  OutDataType=sfix(16)  OutScaling=2^0
  wires:
  C Function Call [ecanFunctions.c]/1 -> Demux/1
  Demux/1 -> Extract Bits2/1, Compare To Zero/1
  Demux/3 -> Decompose uint64/2(high-order uint1)
  Demux/4 -> Extract Bits/1, Extract Bits1/1
  Data Type Conversion/1 -> remote/1
  Demux/2 -> Decompose uint64/1(low-order uint32)
  Extract Bits/1 -> Data Type Conversion/1
  Decompose uint64/1(uint8 array) -> data/1
  Extract Bits2/1 -> identifier/1
  Compare To Zero/1 -> new/1
  Extract Bits1/1 -> size/1

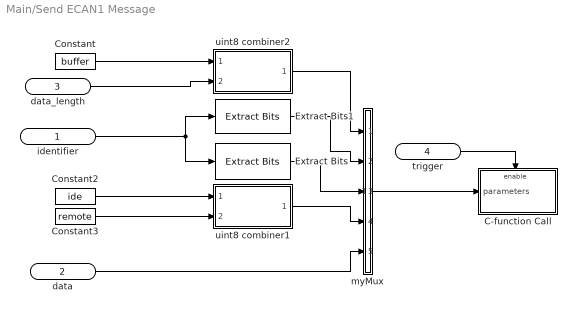
== system Main/Send ECAN1 Message ==
  identifier : Inport  OutDataType=sfix(16)  OutScaling=2^0
  data : Inport  Port=2  OutDataType=sfix(16)  OutScaling=2^0
  data_length : Inport  Port=3  OutDataType=sfix(16)  OutScaling=2^0
  trigger : Inport  Port=4  OutDataType=sfix(16)  OutScaling=2^0
  C-function Call : Subsystem
  Constant : Constant  Value=buffer  OutDataTypeMode=uint8  OutDataType=sfix(16)  OutScaling=2^0  OutDataTypeStr=uint8
  Constant2 : Constant  Value=ide  OutDataTypeMode=uint8  OutDataType=sfix(16)  OutScaling=2^0  OutDataTypeStr=uint8
  Constant3 : Constant  Value=remote  OutDataTypeMode=uint8  OutDataType=sfix(16)  OutScaling=2^0  OutDataTypeStr=uint8
  Extract Bits : simulink/Logic and Bit Operations/Extract Bits  SystemSampleTime=-1  bitsToExtract=Upper half  numBits=8  bitIdxRange=[0 7]  outScalingMode=Treat bit field as an integer
  Extract Bits1 : simulink/Logic and Bit Operations/Extract Bits  SystemSampleTime=-1  bitsToExtract=Lower half  numBits=8  bitIdxRange=[0 7]  outScalingMode=Preserve fixed-point scaling
  myMux : Stateflow chart  TreatAsAtomicUnit=on
  uint8 combiner1 : Subsystem
  uint8 combiner2 : Subsystem
  wires:
  trigger/1 -> C-function Call/Enable
  Constant/1 -> uint8 combiner2/1(high-order)
  data_length/1 -> uint8 combiner2/2(low-order)
  identifier/1 -> Extract Bits1/1, Extract Bits/1
  Constant3/1 -> uint8 combiner1/2(low-order)
  Constant2/1 -> uint8 combiner1/1(high-order)
  myMux/1(y) -> C-function Call/1(parameters)
  uint8 combiner2/1(combined) -> myMux/1(u1)
  Extract Bits/1 -> myMux/3(u3)
  Extract Bits1/1 -> myMux/2(u2)
  uint8 combiner1/1(combined) -> myMux/4(u4)
  data/1 -> myMux/5(u5)

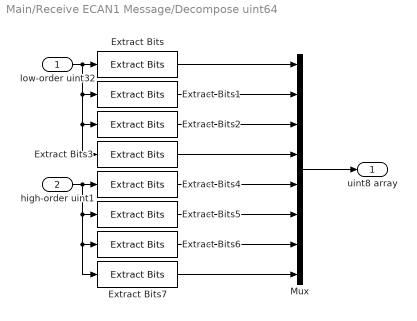
== system Main/Receive ECAN1 Message/Decompose uint64 ==
  low-order uint32 : Inport  OutDataType=sfix(16)  OutScaling=2^0
  high-order uint1 : Inport  Port=2  OutDataType=sfix(16)  OutScaling=2^0
  Extract Bits : simulink/Logic and Bit Operations/Extract Bits  SystemSampleTime=-1  bitsToExtract=Range of bits  numBits=8  bitIdxRange=[0 7]  outScalingMode=Treat bit field as an integer
  Extract Bits1 : simulink/Logic and Bit Operations/Extract Bits  SystemSampleTime=-1  bitsToExtract=Range of bits  numBits=8  bitIdxRange=[8 15]  outScalingMode=Treat bit field as an integer
  Extract Bits2 : simulink/Logic and Bit Operations/Extract Bits  SystemSampleTime=-1  bitsToExtract=Range of bits  numBits=8  bitIdxRange=[16 23]  outScalingMode=Treat bit field as an integer
  Extract Bits3 : simulink/Logic and Bit Operations/Extract Bits  SystemSampleTime=-1  bitsToExtract=Range of bits  numBits=8  bitIdxRange=[24 31]  outScalingMode=Treat bit field as an integer
  Extract Bits4 : simulink/Logic and Bit Operations/Extract Bits  SystemSampleTime=-1  bitsToExtract=Range of bits  numBits=8  bitIdxRange=[0 7]  outScalingMode=Treat bit field as an integer
  Extract Bits5 : simulink/Logic and Bit Operations/Extract Bits  SystemSampleTime=-1  bitsToExtract=Range of bits  numBits=8  bitIdxRange=[8 15]  outScalingMode=Treat bit field as an integer
  Extract Bits6 : simulink/Logic and Bit Operations/Extract Bits  SystemSampleTime=-1  bitsToExtract=Range of bits  numBits=8  bitIdxRange=[16 23]  outScalingMode=Treat bit field as an integer
  Extract Bits7 : simulink/Logic and Bit Operations/Extract Bits  SystemSampleTime=-1  bitsToExtract=Range of bits  numBits=8  bitIdxRange=[24 31]  outScalingMode=Treat bit field as an integer
  Mux : Mux  Inputs=8
  uint8 array : Outport  OutDataType=sfix(16)  OutScaling=2^0
  wires:
  low-order uint32/1 -> Extract Bits/1, Extract Bits1/1, Extract Bits2/1, Extract Bits3/1
  Mux/1 -> uint8 array/1
  high-order uint1/1 -> Extract Bits4/1, Extract Bits5/1, Extract Bits6/1, Extract Bits7/1
  Extract Bits/1 -> Mux/1
  Extract Bits7/1 -> Mux/8
  Extract Bits1/1 -> Mux/2
  Extract Bits2/1 -> Mux/3
  Extract Bits3/1 -> Mux/4
  Extract Bits4/1 -> Mux/5
  Extract Bits5/1 -> Mux/6
  Extract Bits6/1 -> Mux/7

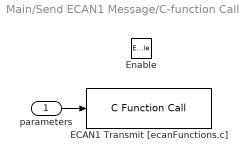
== system Main/Send ECAN1 Message/C-function Call ==
  parameters : Inport  OutDataType=sfix(16)  OutScaling=2^0
  Enable : EnablePort
  ECAN1 Transmit [ecanFunctions.c] : dsPICdrivers/OTHERS/C Function Call  Tag=dsPIC_dsPIC_CFunctionCall  fctName='ecan1_buffered_transmit_matlab'  INPUT_SIZE=8  INPUT1=uint16  INPUT2=--  INPUT3=--  OUTPUT_SIZE=1  OUTPUT1=--  SampleTime=c_func_sample_time  InputType=[ 4 ]  OutputType=[ ]  FctDeclaration=extern void ecan1_buffered_transmit_matlab(uint16_T* u1);  FctCall=ecan1_buffered_transmit_matlab(*%u1);  OrderingInOutPopup=None
  wires:
  parameters/1 -> ECAN1 Transmit [ecanFunctions.c]/1

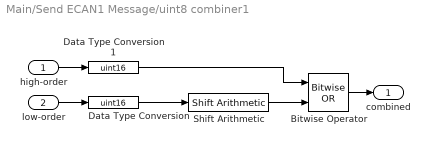
== system Main/Send ECAN1 Message/uint8 combiner1 ==
  high-order : Inport  OutDataType=sfix(16)  OutScaling=2^0
  low-order : Inport  Port=2  OutDataType=sfix(16)  OutScaling=2^0
  Bitwise Operator : simulink/Logic and Bit Operations/Bitwise Operator  logicop=OR  UseBitMask=off  NumInputPorts=2  BitMask=bin2dec('11011001')  BitMaskRealWorld=Stored Integer
  Data Type Conversion : DataTypeConversion  OutDataTypeMode=uint16  OutDataType=sfix(16)  OutScaling=2^0  OutDataTypeStr=uint16
  Data Type Conversion1 : DataTypeConversion  OutDataTypeMode=uint16  OutDataType=sfix(16)  OutScaling=2^0  OutDataTypeStr=uint16
  Shift Arithmetic : simulink/Logic and Bit Operations/Shift Arithmetic  SystemSampleTime=-1  nBitShiftRight=-8  nBinPtShiftRight=0
  combined : Outport  OutDataType=sfix(16)  OutScaling=2^0
  wires:
  low-order/1 -> Data Type Conversion/1
  Bitwise Operator/1 -> combined/1
  high-order/1 -> Data Type Conversion1/1
  Shift Arithmetic/1 -> Bitwise Operator/2
  Data Type Conversion/1 -> Shift Arithmetic/1
  Data Type Conversion1/1 -> Bitwise Operator/1

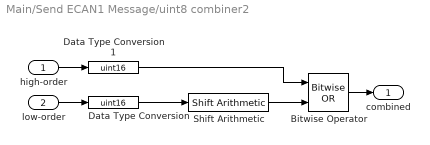
== system Main/Send ECAN1 Message/uint8 combiner2 ==
  high-order : Inport  OutDataType=sfix(16)  OutScaling=2^0
  low-order : Inport  Port=2  OutDataType=sfix(16)  OutScaling=2^0
  Bitwise Operator : simulink/Logic and Bit Operations/Bitwise Operator  logicop=OR  UseBitMask=off  NumInputPorts=2  BitMask=bin2dec('11011001')  BitMaskRealWorld=Stored Integer
  Data Type Conversion : DataTypeConversion  OutDataTypeMode=uint16  OutDataType=sfix(16)  OutScaling=2^0  OutDataTypeStr=uint16
  Data Type Conversion1 : DataTypeConversion  OutDataTypeMode=uint16  OutDataType=sfix(16)  OutScaling=2^0  OutDataTypeStr=uint16
  Shift Arithmetic : simulink/Logic and Bit Operations/Shift Arithmetic  SystemSampleTime=-1  nBitShiftRight=-8  nBinPtShiftRight=0
  combined : Outport  OutDataType=sfix(16)  OutScaling=2^0
  wires:
  Data Type Conversion1/1 -> Bitwise Operator/1
  Data Type Conversion/1 -> Shift Arithmetic/1
  Shift Arithmetic/1 -> Bitwise Operator/2
  high-order/1 -> Data Type Conversion1/1
  Bitwise Operator/1 -> combined/1
  low-order/1 -> Data Type Conversion/1

== matlab function Send ECAN1 Message/myMux ==
  data: u1 input double; y output double; u2 input double; u3 input double; u4 input double; u5 input double
function y = myMux(u1, u2, u3, u4, u5)
u5_u16 = uint16(u5);
y = uint16([u1(1); u2(1); u3(1); u4(1); 0; 0; 0; 0;]);

len = length(u5);
if len > 1
    y(5) = bitor(bitshift(u5_u16(1),8),u5_u16(2));
elseif len > 0
    y(5) = u5_u16(1);
end
if len > 3
    y(6) = bitor(bitshift(u5_u16(3),8),u5_u16(4));
elseif len > 2
    y(6) = u5_u16(3);
end
if len > 5
    y(7) = bitor(bitshift(u5_u16(5),8),u5_u16(6));
elseif len > 4
    y(7) = u5_u16(5);
end
if len > 7
    y(8) = bitor(bitshift(u5_u16(7),8),u5_u16(8));
elseif len > 6
    y(8) = u5_u16(7);
end
